simulink model "buck_circuito_completo"  (R2026a)
settings: Solver=ode23t  StopTime=12e-3  MaxStep=1e-6  RelTol=1e-4
PreLoadFcn:
  | circuito_completo_parametros;
values from neighbouring files (symbols this model uses):
  ADC_A_UV = 389000    [circuito_completo_parametros.m]
  ADC_B_X1E5 = 8251    [circuito_completo_parametros.m]
  D_FIXO_PERMIL = 500    [circuito_completo_parametros.m]
  MODO = 1    [circuito_completo.m]    (also in circuito_completo_parametros.m = 0)
  R_pot = 46.6    [circuito_completo_parametros.m]
  T_KEY = 0    [circuito_completo.m]    (also in circuito_completo_parametros.m = 0.001)
  Ts = 1e-4    (= 0.0001)    [circuito_completo_parametros.m]    (also in etapa01_referencia.m; etapa02_projeto_buck.m; etapa02_simulink.m; etapa03_projeto_ccs.m)
libraries: fl_lib x69, nesl_utility x15, ee_lib x10, simulink x1
(part 2 of 2)

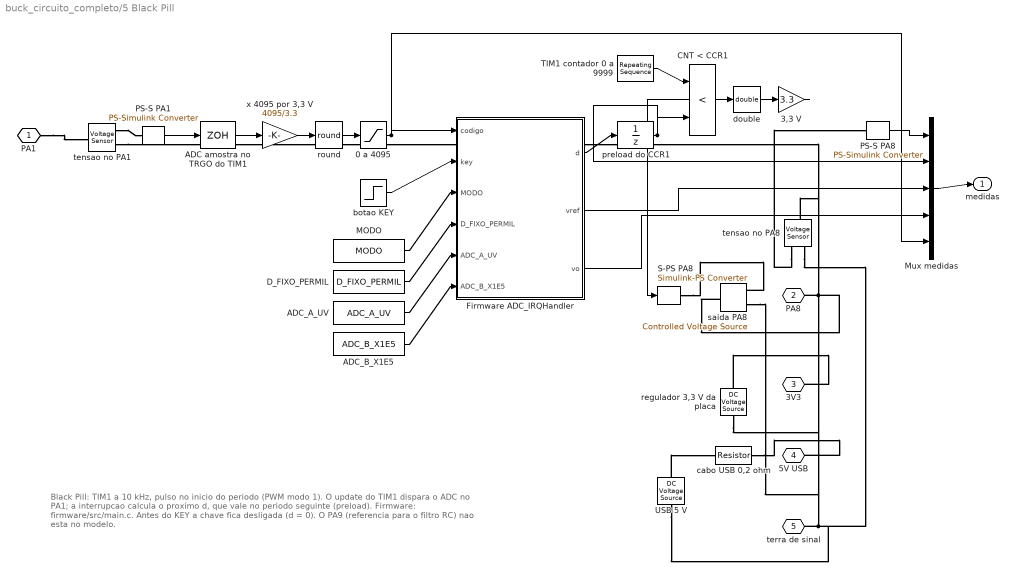
== system buck_circuito_completo/5 Black Pill ==
  note: Black Pill: TIM1 a 10 kHz, pulso no inicio do periodo (PWM modo 1). O update do TIM1 dispara o ADC no PA1;
      | a interrupcao calcula o proximo d, que vale no periodo seguinte (preload). Firmware: firmware/src/main.c.
      | Antes do KEY a chave fica desligada (d = 0). O PA9 (referencia para o filtro RC) nao esta no modelo.
  0 a 4095 : Saturate  UpperLimit=4095  LowerLimit=0
  3,3 V : Gain  Gain=3.3
  ADC amostra no TRGO do TIM1 : ZeroOrderHold  SampleTime=Ts
  ADC_A_UV : Constant  Value=ADC_A_UV
  ADC_B_X1E5 : Constant  Value=ADC_B_X1E5
  CNT < CCR1 : RelationalOperator  Operator=<  OutDataTypeStr=boolean  RndMeth=Simplest  InputSameDT=off
  D_FIXO_PERMIL : Constant  Value=D_FIXO_PERMIL
  Firmware ADC_IRQHandler : MATLAB Function  TreatAsAtomicUnit=on
  MODO : Constant  Value=MODO
  Mux medidas : Mux  Inputs=5
  PS-S PA1 : nesl_utility/PS-Simulink Converter  PhysicalDomain=network_engine_domain  SubClassName=ps_output  LeftPortType=input  RightPortType=output  PseudoPeriodic=off  Frequencies=[]  VectorFormat=inherit  Unit=V  AffineConversion=off
  PS-S PA8 : nesl_utility/PS-Simulink Converter  PhysicalDomain=network_engine_domain  SubClassName=ps_output  LeftPortType=input  RightPortType=output  PseudoPeriodic=off  Frequencies=[]  VectorFormat=inherit  Unit=V  AffineConversion=off
  S-PS PA8 : nesl_utility/Simulink-PS Converter  PhysicalDomain=network_engine_domain  SubClassName=ps_input  LeftPortType=input  RightPortType=output  PseudoPeriodic=off  Frequencies=[]  NoiseDistribution=none  NoiseParameters=[]  Unit=V  AffineConversion=off  FilteringAndDerivatives=zero  SimscapeFilterOrder=1  InputFilterTimeConstant=0.001  UdotUserProvided=0
  TIM1 contador 0 a 9999 : simulink/Sources/Repeating Sequence  rep_seq_t=[0 Ts]  rep_seq_y=[0 1]
  USB 5 V : fl_lib/Electrical/Electrical Sources/DC Voltage Source  v0=5 V
  botao KEY : Step  Time=T_KEY  SampleTime=Ts
  cabo USB 0,2 ohm : fl_lib/Electrical/Electrical Elements/Resistor  R=0.2 Ohm  i_specify=off  i_priority=None  i=0 A  i_nominal_specify=off  i_nominal_value=1  i_nominal_unit=A  v_specify=off  v_priority=None  v=0 V  v_nominal_specify=off  v_nominal_value=1  v_nominal_unit=V
  double : DataTypeConversion  OutDataTypeStr=double  SaturateOnIntegerOverflow=off  RndMeth=Floor
  preload do CCR1 : UnitDelay  SampleTime=Ts
  regulador 3,3 V da placa : fl_lib/Electrical/Electrical Sources/DC Voltage Source  v0=3.3 V
  round : Rounding  Operator=round
  saida PA8 : fl_lib/Electrical/Electrical Sources/Controlled Voltage Source
  tensao no PA1 : fl_lib/Electrical/Electrical Sensors/Voltage Sensor
  tensao no PA8 : fl_lib/Electrical/Electrical Sensors/Voltage Sensor
  x 4095 por 3,3 V : Gain  Gain=4095/3.3
  PA1 : PMIOPort  Side=Left
  PA8 : PMIOPort  Port=2  Side=Right
  3V3 : PMIOPort  Port=3  Side=Right
  5V USB : PMIOPort  Port=4  Side=Right
  terra de sinal : PMIOPort  Port=5  Side=Right
  medidas : Outport
  wires:
  PS-S PA1/1 -> ADC amostra no TRGO do TIM1/1
  ADC amostra no TRGO do TIM1/1 -> x 4095 por 3,3 V/1
  x 4095 por 3,3 V/1 -> round/1
  round/1 -> 0 a 4095/1
  0 a 4095/1 -> Firmware ADC_IRQHandler/1(codigo), Mux medidas/5
  botao KEY/1 -> Firmware ADC_IRQHandler/2(key)
  MODO/1 -> Firmware ADC_IRQHandler/3(MODO)
  D_FIXO_PERMIL/1 -> Firmware ADC_IRQHandler/4(D_FIXO_PERMIL)
  ADC_A_UV/1 -> Firmware ADC_IRQHandler/5(ADC_A_UV)
  ADC_B_X1E5/1 -> Firmware ADC_IRQHandler/6(ADC_B_X1E5)
  Firmware ADC_IRQHandler/1(d) -> preload do CCR1/1
  TIM1 contador 0 a 9999/1 -> CNT < CCR1/1
  preload do CCR1/1 -> CNT < CCR1/2, Mux medidas/2
  CNT < CCR1/1 -> double/1
  double/1 -> 3,3 V/1
  3,3 V/1 -> S-PS PA8/1
  Mux medidas/1 -> medidas/1
  PS-S PA8/1 -> Mux medidas/1
  Firmware ADC_IRQHandler/2(vref) -> Mux medidas/3
  Firmware ADC_IRQHandler/3(vo) -> Mux medidas/4
  connections:
  PA1/RConn1 -- tensao no PA1/LConn1
  tensao no PA1/RConn2 -- saida PA8/RConn2 -- regulador 3,3 V da placa/RConn1 -- USB 5 V/RConn1 -- terra de sinal/RConn1 -- tensao no PA8/RConn2
  tensao no PA1/RConn1 -- PS-S PA1/LConn1
  S-PS PA8/RConn1 -- saida PA8/RConn1
  PA8/RConn1 -- saida PA8/LConn1 -- tensao no PA8/LConn1
  regulador 3,3 V da placa/LConn1 -- 3V3/RConn1
  USB 5 V/LConn1 -- cabo USB 0,2 ohm/LConn1
  cabo USB 0,2 ohm/RConn1 -- 5V USB/RConn1
  tensao no PA8/RConn1 -- PS-S PA8/LConn1

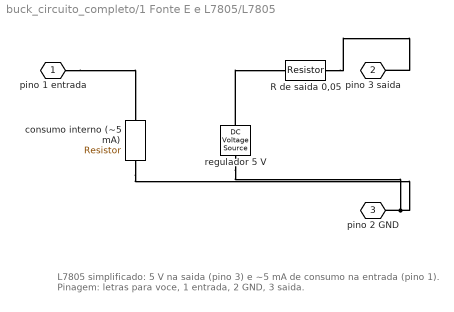
== system buck_circuito_completo/1 Fonte E e L7805/L7805 ==
  note: L7805 simplificado: 5 V na saida (pino 3) e ~5 mA de consumo na entrada (pino 1).
      | Pinagem: letras para voce, 1 entrada, 2 GND, 3 saida.
  R de saida 0,05 : fl_lib/Electrical/Electrical Elements/Resistor  R=0.05 Ohm  i_specify=off  i_priority=None  i=0 A  i_nominal_specify=off  i_nominal_value=1  i_nominal_unit=A  v_specify=off  v_priority=None  v=0 V  v_nominal_specify=off  v_nominal_value=1  v_nominal_unit=V
  consumo interno (~5 mA) : fl_lib/Electrical/Electrical Elements/Resistor  R=4.7e3 Ohm  i_specify=off  i_priority=None  i=0 A  i_nominal_specify=off  i_nominal_value=1  i_nominal_unit=A  v_specify=off  v_priority=None  v=0 V  v_nominal_specify=off  v_nominal_value=1  v_nominal_unit=V
  regulador 5 V : fl_lib/Electrical/Electrical Sources/DC Voltage Source  v0=5 V
  pino 1 entrada : PMIOPort  Side=Left
  pino 3 saida : PMIOPort  Port=2  Side=Right
  pino 2 GND : PMIOPort  Port=3  Side=Right
  connections:
  pino 1 entrada/RConn1 -- consumo interno (~5 mA)/LConn1
  pino 2 GND/RConn1 -- consumo interno (~5 mA)/RConn1 -- regulador 5 V/RConn1
  regulador 5 V/LConn1 -- R de saida 0,05/LConn1
  R de saida 0,05/RConn1 -- pino 3 saida/RConn1

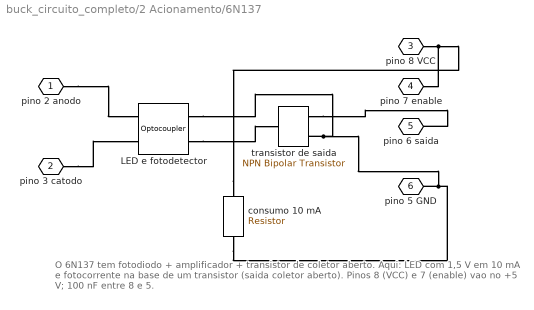
== system buck_circuito_completo/2 Acionamento/6N137 ==
  note: O 6N137 tem fotodiodo + amplificador + transistor de coletor aberto.
      | Aqui: LED com 1,5 V em 10 mA e fotocorrente na base de um transistor (saida coletor aberto).
      | Pinos 8 (VCC) e 7 (enable) vao no +5 V; 100 nF entre 8 e 5.
  LED e fotodetector : ee_lib/Semiconductors & Converters/Optocoupler  CTR=0.01  prmExp=1  I12=[1e-3 10e-3] A  V12=[1.3 1.5] V  IS=1e-10 A  ec=2  RS=0.1 Ohm  Tmeas=25 degC  C_param=1  CJ=5 pF  CJ0=5 pF  VJ=1 V  Mgrad=0.5  Vvec=[.1, 10, 100] V  Cvec=[3.5, 1, .4] pF  FC=0.5  T_param=1  IS_T2=1.8e-8 A  I1_T2=0.029 A  V1_T2=1.05 V  Tmeas2=125 degC  EG_param=1  EG=1.11 eV  XTI_param=1  XTI=3  Tdevice=25 degC  i_specify=off  i_priority=None  i=0 A  i_nominal_specify=off  i_nominal_value=1  i_nominal_unit=A  v_specify=off  v_priority=None  v=0 V  v_nominal_specify=off  v_nominal_value=1  v_nominal_unit=V  v_capacitor_specify=off  v_capacitor_priority=None  v_capacitor=0 V  v_capacitor_nominal_specify=off  v_capacitor_nominal_value=1  v_capacitor_nominal_unit=V  thermal_network_parameterization=ee.enum.thermalNetworkTopology.junctionCase  Rth=[0, 10] K/W  Rth_Cauer=[1, 3, 10] K/W  Rth_Foster=[.08, .14, .22, .16] K/W  thermal_mass_parameterization=ee.enum.thermalNetwork.timeconstant  thermal_mass=[0, 1] J/K  thermal_mass_Cauer=[.1, .3, 1] J/K  thermal_mass_Foster=[.001, .005, .05, .5] J/K  thermal_time_constant=[0, 10] s  thermal_time_constant_Cauer=[1, 3, 10] s  thermal_time_constant_Foster=[7e-05, .0007, .01, .08] s  thermal_mass_initial_temperatures=[25, 25] degC  thermal_mass_initial_temperatures_Cauer=[25, 25, 25] degC  Tvec_initial_Foster=[25, 25, 25, 25] degC  i_capacitor_specify=off  i_capacitor_priority=High  i_capacitor=0 A  i_capacitor_nominal_specify=off  i_capacitor_nominal_value=1  i_capacitor_nominal_unit=A
  consumo 10 mA : fl_lib/Electrical/Electrical Elements/Resistor  R=500 Ohm  i_specify=off  i_priority=None  i=0 A  i_nominal_specify=off  i_nominal_value=1  i_nominal_unit=A  v_specify=off  v_priority=None  v=0 V  v_nominal_specify=off  v_nominal_value=1  v_nominal_unit=V
  transistor de saida : ee_lib/Semiconductors & Converters/NPN Bipolar Transistor  parameterization=1  BF=100  IS=1e-14 A  VAF=200 V  hfe=100  hoe=50e-6 1/Ohm  Ic_h=1 mA  Vce_h=5 V  V1=0.55 V  I1=0.5 mA  BR=1  Tmeas=25 degC  RC=0.01 Ohm  RE=1e-4 Ohm  RB=1 Ohm  C_BC=5 pF  C_BE=5 pF  TF=0 us  TR=0 us  prmDatasheet=1  prmEquCoeff=1  hfe_T2=125  XTB=0  V1_T2=0.45 V  I1_T2=0.5 mA  Tmeas2=125 degC  EG=1.11 eV  XTI=3  TdeviceDatasheet=25 degC  TdeviceEquCoeff=25 degC  ec=1  ib_specify=off  ib_priority=None  ib=0 A  ib_nominal_specify=off  ib_nominal_value=1  ib_nominal_unit=A  ic_specify=off  ic_priority=None  ic=0 A  ic_nominal_specify=off  ic_nominal_value=1  ic_nominal_unit=A  vce_specify=off  vce_priority=None  vce=0 V  vce_nominal_specify=off  vce_nominal_value=1  vce_nominal_unit=V  vbe_specify=off  vbe_priority=None  vbe=0 V  vbe_nominal_specify=off  vbe_nominal_value=1  vbe_nominal_unit=V  Qbc_specify=off  Qbc_priority=High  Qbc=0 C  Qbc_nominal_specify=off  Qbc_nominal_value=1  Qbc_nominal_unit=uC  Qbe_specify=off  Qbe_priority=High  Qbe=0 C  Qbe_nominal_specify=off  Qbe_nominal_value=1  Qbe_nominal_unit=uC  thermal_network_parameterization=ee.enum.thermalNetworkTopology.junctionCase  Rth=[0, 10] K/W  Rth_Cauer=[1, 3, 10] K/W  Rth_Foster=[.08, .14, .22, .16] K/W  thermal_mass_parameterization=ee.enum.thermalNetwork.timeconstant  thermal_mass=[0, 1] J/K  thermal_mass_Cauer=[.1, .3, 1] J/K  thermal_mass_Foster=[.001, .005, .05, .5] J/K  thermal_time_constant=[0, 10] s  thermal_time_constant_Cauer=[1, 3, 10] s  thermal_time_constant_Foster=[7e-05, .0007, .01, .08] s  thermal_mass_initial_temperatures=[25, 25] degC  thermal_mass_initial_temperatures_Cauer=[25, 25, 25] degC  Tvec_initial_Foster=[25, 25, 25, 25] degC
  pino 2 anodo : PMIOPort  Side=Left
  pino 3 catodo : PMIOPort  Port=2  Side=Left
  pino 8 VCC : PMIOPort  Port=3  Side=Right
  pino 7 enable : PMIOPort  Port=4  Side=Right
  pino 6 saida : PMIOPort  Port=5  Side=Right
  pino 5 GND : PMIOPort  Port=6  Side=Right
  connections:
  consumo 10 mA/LConn1 -- pino 8 VCC/RConn1 -- pino 7 enable/RConn1
  pino 5 GND/RConn1 -- consumo 10 mA/RConn1 -- LED e fotodetector/RConn1 -- transistor de saida/RConn2
  pino 2 anodo/RConn1 -- LED e fotodetector/LConn1
  pino 3 catodo/RConn1 -- LED e fotodetector/LConn2
  LED e fotodetector/RConn2 -- transistor de saida/LConn1
  transistor de saida/RConn1 -- pino 6 saida/RConn1

== matlab function buck_circuito_completo/5 Black Pill/Firmware ADC_IRQHandler ==
  data: codigo input; d output; key input; MODO input; D_FIXO_PERMIL input; ADC_A_UV input; ADC_B_X1E5 input; vref output; vo output
function [d, vref, vo] = firmware(codigo, key, MODO, D_FIXO_PERMIL, ADC_A_UV, ADC_B_X1E5)
% Mesma conta da ADC_IRQHandler (firmware/src/main.c), em inteiros.
% Saidas: d (0 a 1), vref [V] do Sinal 1, vo [V] reconstruido do ADC.
persistent k n_acima falha
if isempty(k), k = 0; n_acima = 0; falha = false; end

% Vo = (v_ADC - A)/B
v_uv  = floor(codigo*33000/4095)*100;
vo_mv = fix((v_uv - ADC_A_UV)*100/ADC_B_X1E5);

% Referencia do Sinal 1 [mV]: 400 amostras por ciclo (40 ms)
vref_mv = referencia_mv(k);
k = k + 1; if k == 400, k = 0; end

% Protecao: Vo > 25 V por 20 amostras desliga a chave
if vo_mv > 25000, n_acima = n_acima + 1; else, n_acima = 0; end
if n_acima >= 20, falha = true; end

% Razao ciclica em contagens do TIM1 (0 a 10000)
cont = 0;
if key > 0.5 && ~falha
    if MODO == 1
        cont = min(10000, floor(vref_mv*100/240));   % d = vref/24 V
    else
        cont = D_FIXO_PERMIL*10;
    end
    % Etapas 8 e 9: o controlador entra aqui, cont = f(vref_mv, vo_mv)
end
d = cont/10000; vref = vref_mv/1000; vo = vo_mv/1000;
end

function v = referencia_mv(k)
vmed = 12000; dv = 6000; passo = 600;
if k >= 50 && k < 60,       v = vmed + passo*(k - 50);
elseif k >= 60 && k < 150,  v = vmed + dv;
elseif k >= 150 && k < 160, v = vmed + dv - passo*(k - 150);
elseif k >= 250 && k < 260, v = vmed - passo*(k - 250);
elseif k >= 260 && k < 350, v = vmed - dv;
elseif k >= 350 && k < 360, v = vmed - dv + passo*(k - 350);
else,                       v = vmed;
end
end
